simulink model "mod_mal"  (R2025a)
settings: Solver=ode45  StartTime=0.0  StopTime=20  MaxStep=1e-2  RelTol=1e-3
settings Model: Creator=fabri  LastModifiedBy=fabri

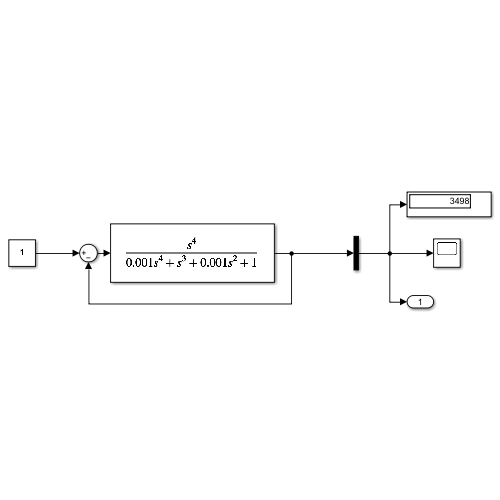
[thumbnail: Simulink's stored preview of the top-level diagram]
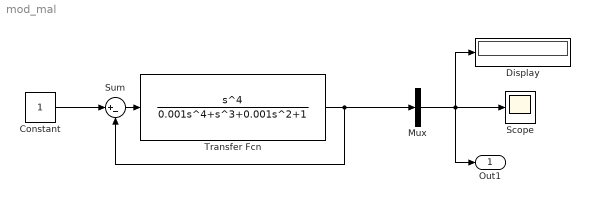
== system mod_mal ==
  Constant : Constant
  Display : Display
  Mux : Mux  Inputs=1
  Scope : Scope
      settings: ActiveDisplayYMinimum=-1456.985150598477  ActiveDisplayYMaximum=6090.7888914953683
  Sum : Sum  Inputs=|+-
  Transfer Fcn : TransferFcn  Numerator=[1 0 0 0 0]  Denominator=[0.001 1 0.001 0 1]
  Out1 : Outport
  wires:
  Sum/1 -> Transfer Fcn/1
  Transfer Fcn/1 -> Mux/1, Sum/2
  Mux/1 -> Scope/1, Out1/1, Display/1
  Constant/1 -> Sum/1
